simulink model "demoOtterUSVHeadingControl"  (R2024a)
settings: Solver=ode4  StartTime=0.0  StopTime=60  FixedStep=0.02  RelTol=1e-3
libraries: mssSimulink x3
settings Model: Creator=thor  LastModifiedBy=thor
settings DebuggingCC: UnconnectedInputMsg=warning  UnconnectedOutputMsg=warning  UnconnectedLineMsg=warning
settings ModelReferenceCC: EnableRefExpFcnMdlSchedulingChecks=on
settings RTWCC: GPUComputeCapability=3.5  DLArmComputeVersion=19.05

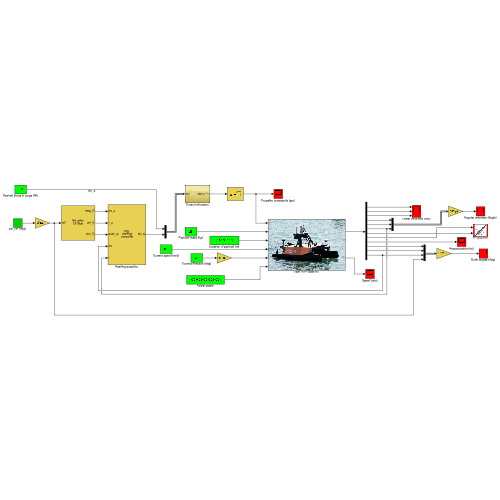
[thumbnail: Simulink's stored preview of the top-level diagram]
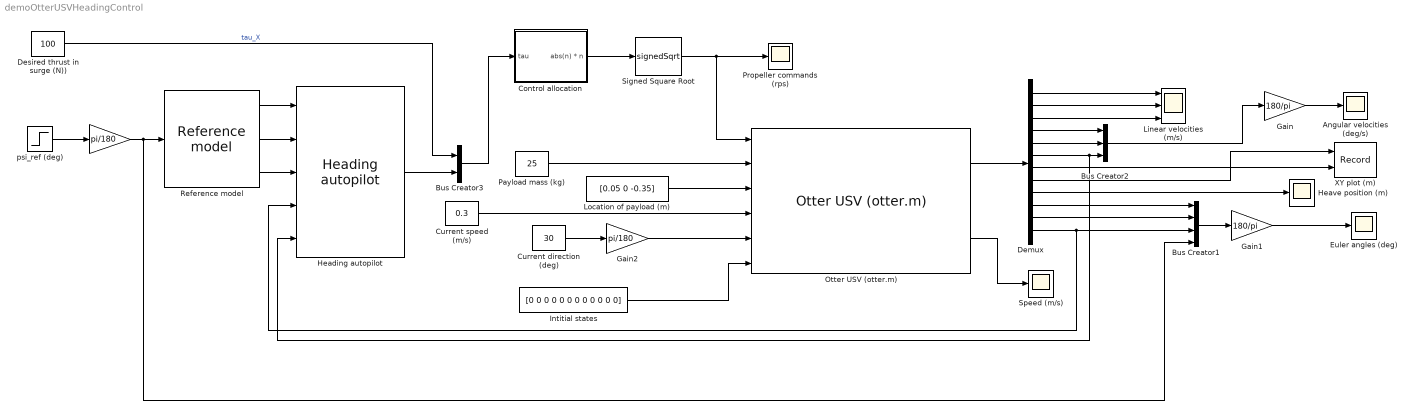
== system demoOtterUSVHeadingControl ==
  " " : Gain  Gain=pi/180
  Angular velocities (deg/s) : Scope
  Bus Creator1 : BusCreator  Inputs=4
  Bus Creator2 : BusCreator  Inputs=3
  Bus Creator3 : BusCreator  Inputs=2
  Control allocation : Subsystem
  Current direction (deg) : Constant  Value=30
  Current speed (m/s) : Constant  Value=0.3
  Demux : Demux  Outputs=12
  Desired thrust in surge (N)) : Constant  Value=100
  Euler angles (deg) : Scope
  Gain : Gain  Gain=180/pi
  Gain1 : Gain  Gain=180/pi
  Gain2 : Gain  Gain=pi/180
  "Heading autopilot " : mssSimulink/Control/Autopilots/Heading autopilot  T_nomoto=1.0  K_nomoto=0.0242  Kp=258.75  Td=0.64  Ti=4
  Heave position (m) : Scope
  Intitial states : Constant  Value=[0 0 0 0 0 0 0 0 0 0 0 0]
  Linear velocities (m/s) : Scope  NumInputPorts=3
  Location of payload (m) : Constant  Value=[0.05 0 -0.35]
  "Otter USV (otter.m) " : mssSimulink/Marine craft models/Otter USV (otter.m)  SystemSampleTime=-1  VariantActivationTime=update diagram  AllowFlexibleInterface=on  Latency=0  AutoFrameSizeCalculation=off
      link override Transfer Fcn: Denominator=[0.1 1]
      link override Transfer Fcn1: Denominator=[0.1 1]
  Payload mass (kg) : Constant  Value=25
  Propeller commands (rps) : Scope
  Reference model : mssSimulink/Guidance/Reference model  v_max=10  zeta_d=1.0  w_d=0.5
  Signed Square Root : Sqrt  Operator=signedSqrt
  Speed (m/s) : Scope
  XY plot (m) : Record  FileSettingsInternal="{\"entries\":[{\"content\":{\"excelSettings\":{\"content\":{},\"type\":\"Streamout.ExcelSettings\"}},\"type\":\"Streamout.FileSettingStorage\",\"uuid\":\"\"}],\"packageUris\":[\"http:\\/\\/schema.mathworks.com\\/mf0\\/streamout_blocks\\/R2020a\"],\"version\":\"1.0\"}"  Layout=[1 1]  SignalsInternal="{\"entries\":[{\"content\":{\"signals\":[{\"content\":{\"blockPath\":[],\"dimensions\":[1],\"domain\":\"\",\"lineColor\":\"#a2142f\",\"plots\":[ 1 ],\"port\":1,\"sid\":[\"\"],\"signalID\":1,\"signalName\":\"Demux:8\"},\"type\":\"RecordBlkView.Signal\",\"uuid\":\"\"},{\"content\":{\"blockPath\":[],\"dimensions\":[1],\"domain\":\"\",\"lineColor\":\"#139fff\",\"plots\":[ 1 ],\"port\":2,\"sid\":[\"\"],\"signalID\":2,\"signalName\":\"Demux:7\"},\"type\":\"RecordBlkView.Signal\",\"uuid\":\"\"}]},\"type\":\"RecordBlkView.InputSignals\",\"uuid\":\"\"}],\"packageUris\":[\"http:\\/\\/schema.mathworks.com\\/mf0\\/streamout_blocks\\/R2020a\"],\"version\":\"1.0\"}"  VisualizationBindings="{\"xyplotplugin\":{\"info\":[{\"series\":[{\"bindingParametersList\":[{\"parameter\":\"X-Axis\",\"signalID\":1,\"signalName\":\"Demux:8\"},{\"parameter\":\"Y-Axis\",\"signalID\":2,\"signalName\":\"Demux:7\"}],\"seriesID\":0}],\"subplotID\":1}]}}"  CompatibilityTag=XY  st=-1
  psi_ref (deg) : Step  Time=30  Before=20  After=0
  wires:
  Demux/8 -> XY plot (m)/1
  Demux/7 -> XY plot (m)/2
  Demux/1 -> Linear velocities (m/s)/1
  Demux/2 -> Linear velocities (m/s)/2
  Demux/3 -> Linear velocities (m/s)/3
  Demux/10 -> Bus Creator1/1
  Demux/11 -> Bus Creator1/2
  Demux/4 -> Bus Creator2/1
  Demux/5 -> Bus Creator2/2
  Bus Creator2/1 -> Gain/1
  Demux/9 -> Heave position (m)/1
  Payload mass (kg)/1 -> "Otter USV (otter.m) "/2
  Location of payload (m)/1 -> "Otter USV (otter.m) "/3
  Current speed (m/s)/1 -> "Otter USV (otter.m) "/4
  Current direction (deg)/1 -> Gain2/1
  Intitial states/1 -> "Otter USV (otter.m) "/6
  "Otter USV (otter.m) "/1 -> Demux/1
  "Otter USV (otter.m) "/2 -> Speed (m/s)/1
  Gain/1 -> Angular velocities (deg/s)/1
  Gain1/1 -> Euler angles (deg)/1
  Gain2/1 -> "Otter USV (otter.m) "/5
  "Heading autopilot "/1 -> Bus Creator3/2
  Demux/12 -> "Heading autopilot "/4, Bus Creator1/3
  Demux/6 -> "Heading autopilot "/5, Bus Creator2/3
  Desired thrust in surge (N))/1 -> Bus Creator3/1  "tau_X"
  Reference model/1 -> "Heading autopilot "/1
  Reference model/2 -> "Heading autopilot "/2
  Reference model/3 -> "Heading autopilot "/3
  " "/1 -> Bus Creator1/4, Reference model/1
  Bus Creator1/1 -> Gain1/1
  Signed Square Root/1 -> "Otter USV (otter.m) "/1, Propeller commands (rps)/1
  Bus Creator3/1 -> Control allocation/1(tau)
  Control allocation/1(abs(n) * n) -> Signed Square Root/1
  psi_ref (deg)/1 -> " "/1

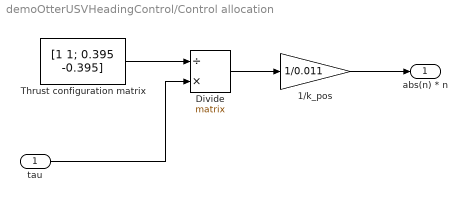
== system demoOtterUSVHeadingControl/Control allocation ==
  tau : Inport
  1/k_pos : Gain  Gain=1/0.011
  Divide : Product  Inputs=/*  Multiplication=Matrix(*)
  Thrust configuration matrix : Constant  Value=[1 1; 0.395 -0.395]
  abs(n) * n : Outport
  wires:
  tau/1 -> Divide/2
  Divide/1 -> 1/k_pos/1
  1/k_pos/1 -> abs(n) * n/1
  Thrust configuration matrix/1 -> Divide/1
